simulink model "Exercise_1_1_model_step_B"  (R2025b)
settings: Solver=VariableStepAuto  StartTime=0.0  StopTime=0.25  RelTol=1e-3
settings Model: Creator=atharvaedake  LastModifiedBy=atharvaedake

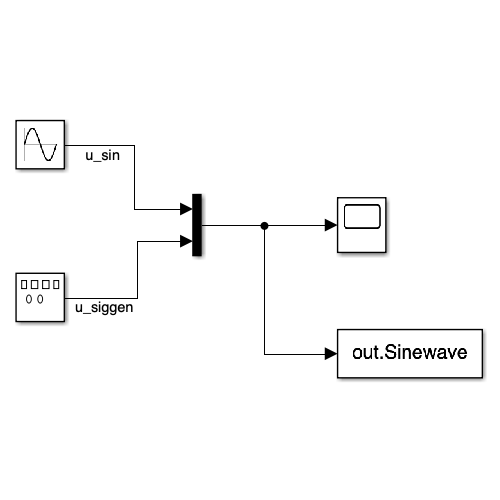
[thumbnail: Simulink's stored preview of the top-level diagram]
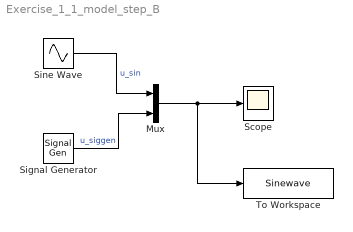
== system Exercise_1_1_model_step_B ==
  Mux : Mux  Inputs=2
  Scope : Scope
      settings: ActiveDisplayYMinimum=-1.0502014869215457E+8  ActiveDisplayYMaximum=1.1923133862478656E+8
  Signal Generator : SignalGenerator  Amplitude=10  Frequency=10
  Sine Wave : Sin  Amplitude=10  Frequency=10*2*pi  SampleTime=0
  To Workspace : ToWorkspace  VariableName=Sinewave  SampleTime=-1
  wires:
  Sine Wave/1 -> Mux/1  "u_sin"
  Signal Generator/1 -> Mux/2  "u_siggen"
  Mux/1 -> To Workspace/1, Scope/1
